simulink model "INC"  (R2020b)
settings: Solver=FixedStepAuto  StartTime=0.0  StopTime=10  FixedStep=1e-2  RelTol=1e-3
libraries: powerlib x1
settings Model: Creator=flocment  LastModifiedBy=bergeslo

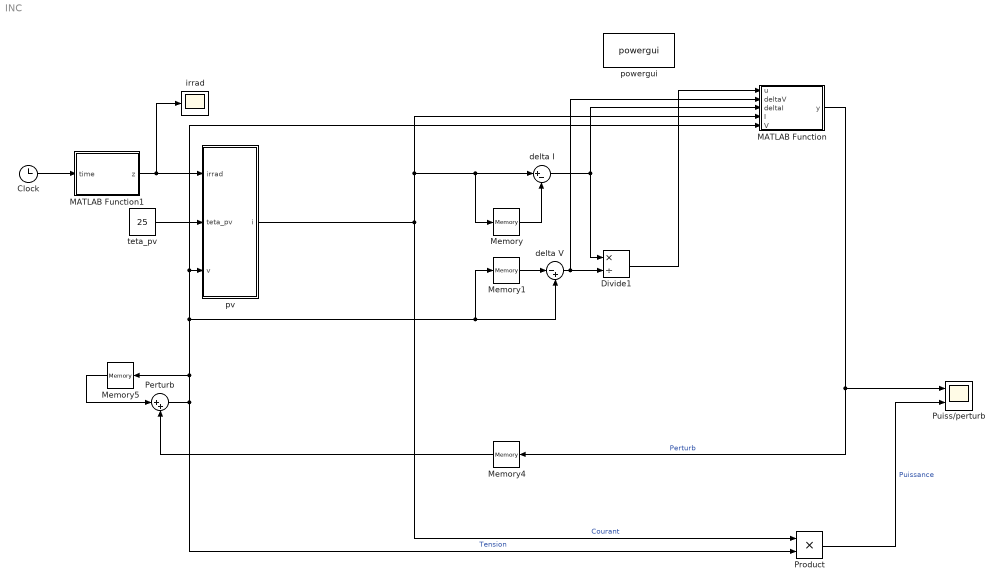
== system INC ==
  Clock : Clock
  Divide1 : Product  Inputs=*/
  MATLAB Function : MATLAB Function  TreatAsAtomicUnit=on
  MATLAB Function1 : MATLAB Function  TreatAsAtomicUnit=on
  Memory : Memory
  Memory1 : Memory
  Memory4 : Memory
  Memory5 : Memory  InitialCondition=5
  Perturb : Sum  Inputs=|++
  Product : Product
  Puiss/perturb : Scope  NumInputPorts=2
  delta I : Sum  Inputs=|+-
  delta V : Sum  Inputs=|-+
  irrad : Scope
  powergui : powerlib/powergui  Priority=1  SimulationMode=Continuous  SampleTime=50e-6  frequency=60  Iterations=50  frequencyindice=60  Pbase=100e6  ErrMax=1e-4  UnitsV=kV  UnitsW=MW  buscounter=0  FunctionMessages=off  echomessages=off  EnableUseOfTLC=off  CurrentSourceSwitches=off  DisableSnubberDevices=off  DisableRonSwitches=off  DisableVfSwitches=off  DisplayEquations=off  AutomaticDiscreteSolvers=off  SolverType=Tustin/Backward Euler (TBE)  Interpol=off  ExternalGateDelay=off  methode=off  Ts=100  x0status=blocks  SPID=on  SwTol=0  HookPort=off  NonlinearTolerance=1e-4  nMaxIteration=100  ContinueOnMaxIteration=off  RestoreLinks=warning  ResistiveCurrentMeasurement=off  Frange=[0:2:500]  Ylog=off  Xlog=on  ShowGrid=off  save=off  variable=ZData  structure=0  ZoomFFT=off  StartTime=0.0  cycles=1  DisplayStyle=1  fundamental=60  FreqAxis=off  MaxFrequency=1000  frequencyindicesteady=1  RmsSteady=1  display=off
  pv : Subsystem
  teta_pv : Constant  Value=25
  wires:
  teta_pv/1 -> pv/2(teta_pv)
  pv/1(i) -> Memory/1, delta I/1, MATLAB Function/4(I), Product/1  "Courant"
  Memory/1 -> delta I/2
  delta I/1 -> Divide1/1, MATLAB Function/3(deltaI)
  Memory1/1 -> delta V/1
  delta V/1 -> MATLAB Function/2(deltaV), Divide1/2
  Divide1/1 -> MATLAB Function/1(u)
  Memory4/1 -> Perturb/2
  Memory5/1 -> Perturb/1
  Perturb/1 -> Product/2, delta V/2, Memory1/1, MATLAB Function/5(V), pv/3(v), Memory5/1  "Tension"
  MATLAB Function/1(y) -> Puiss/perturb/1, Memory4/1  "Perturb"
  Product/1 -> Puiss/perturb/2  "Puissance"
  Clock/1 -> MATLAB Function1/1(time)
  MATLAB Function1/1(z) -> pv/1(irrad), irrad/1

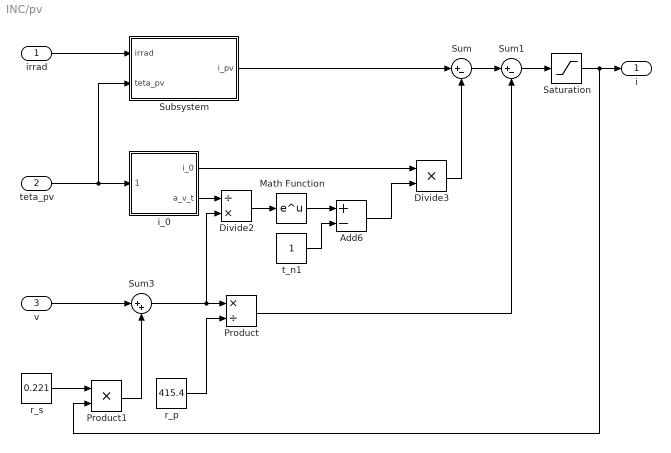
== system INC/pv ==
  irrad : Inport
  teta_pv : Inport  Port=2
  v : Inport  Port=3
  Add6 : Sum  Inputs=+-
  Divide2 : Product  Inputs=/*
  Divide3 : Product  Inputs=**
  Math Function : Math  SaturateOnIntegerOverflow=on
  Product : Product  Inputs=*/
  Product1 : Product
  Saturation : Saturate  UpperLimit=inf  LowerLimit=0
  Subsystem : Subsystem
  Sum : Sum  Inputs=|+-
  Sum1 : Sum  Inputs=|+-
  Sum3 : Sum  Inputs=|++
  i_0 : Subsystem
  r_p : Constant  Value=415.4
  r_s : Constant  Value=0.221
  t_n1 : Constant
  i : Outport
  wires:
  Add6/1 -> Divide3/2
  Sum3/1 -> Divide2/2, Product/1
  Subsystem/1(i_pv) -> Sum/1
  irrad/1 -> Subsystem/1(irrad)
  teta_pv/1 -> Subsystem/2(teta_pv), i_0/1(teta_pv)
  Product1/1 -> Sum3/2
  v/1 -> Sum3/1
  Sum/1 -> Sum1/1
  i_0/1(i_0) -> Divide3/1
  Divide2/1 -> Math Function/1
  i_0/2(a_v_t) -> Divide2/1
  r_p/1 -> Product/2
  r_s/1 -> Product1/1
  t_n1/1 -> Add6/2
  Math Function/1 -> Add6/1
  Sum1/1 -> Saturation/1
  Product/1 -> Sum1/2
  Divide3/1 -> Sum/2
  Saturation/1 -> i/1, Product1/2

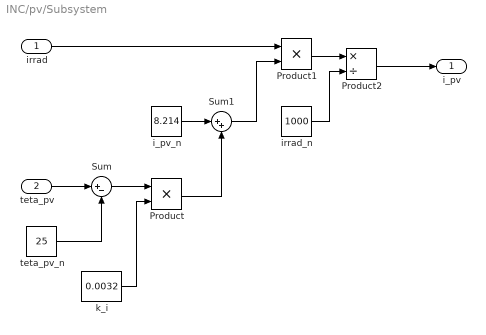
== system INC/pv/Subsystem ==
  irrad : Inport
  teta_pv : Inport  Port=2
  Product : Product
  Product1 : Product
  Product2 : Product  Inputs=*/
  Sum : Sum  Inputs=|+-
  Sum1 : Sum  Inputs=|++
  i_pv_n : Constant  Value=8.214
  irrad_n : Constant  Value=1000
  k_i : Constant  Value=0.0032
  teta_pv_n : Constant  Value=25
  i_pv : Outport
  wires:
  Sum1/1 -> Product1/2
  Product2/1 -> i_pv/1
  teta_pv_n/1 -> Sum/2
  Product1/1 -> Product2/1
  irrad_n/1 -> Product2/2
  Product/1 -> Sum1/2
  i_pv_n/1 -> Sum1/1
  irrad/1 -> Product1/1
  teta_pv/1 -> Sum/1
  k_i/1 -> Product/2
  Sum/1 -> Product/1

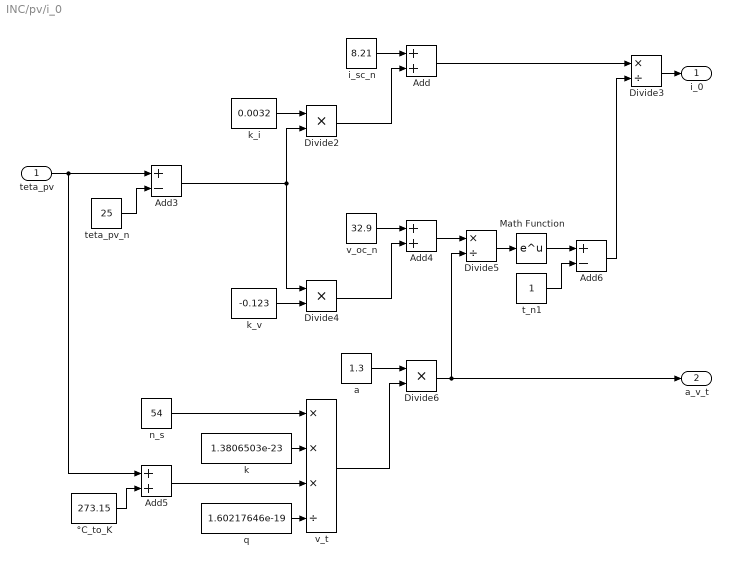
== system INC/pv/i_0 ==
  teta_pv : Inport
  Add : Sum
  Add3 : Sum  Inputs=+-
  Add4 : Sum
  Add5 : Sum
  Add6 : Sum  Inputs=+-
  Divide2 : Product  Inputs=**
  Divide3 : Product  Inputs=*/
  Divide4 : Product  Inputs=**
  Divide5 : Product  Inputs=*/
  Divide6 : Product  Inputs=**
  Math Function : Math  SaturateOnIntegerOverflow=on
  a : Constant  Value=1.3
  i_sc_n : Constant  Value=8.21
  k : Constant  Value=1.3806503e-23
  k_i : Constant  Value=0.0032
  k_v : Constant  Value=-0.123
  n_s : Constant  Value=54
  q : Constant  Value=1.60217646e-19
  t_n1 : Constant
  teta_pv_n : Constant  Value=25
  v_oc_n : Constant  Value=32.9
  v_t : Product  Inputs=***/
  °C_to_K : Constant  Value=273.15
  i_0 : Outport
  a_v_t : Outport  Port=2
  wires:
  Divide3/1 -> i_0/1
  Add4/1 -> Divide5/1
  Add/1 -> Divide3/1
  q/1 -> v_t/4
  k_v/1 -> Divide4/2
  k/1 -> v_t/2
  Divide5/1 -> Math Function/1
  Add5/1 -> v_t/3
  Divide6/1 -> a_v_t/1, Divide5/2
  Math Function/1 -> Add6/1
  Add6/1 -> Divide3/2
  v_t/1 -> Divide6/2
  Add3/1 -> Divide4/1, Divide2/2
  n_s/1 -> v_t/1
  teta_pv/1 -> Add5/1, Add3/1
  Divide4/1 -> Add4/2
  v_oc_n/1 -> Add4/1
  a/1 -> Divide6/1
  t_n1/1 -> Add6/2
  Divide2/1 -> Add/2
  teta_pv_n/1 -> Add3/2
  i_sc_n/1 -> Add/1
  k_i/1 -> Divide2/1
  °C_to_K/1 -> Add5/2

== matlab function INC/MATLAB Function1 ==
  data: time input; z output
function z = fcn(time)
    if time<2
    z=400;
    elseif 2<time && time<5
    z=800;
    else
    z=300;
    end

== matlab function INC/MATLAB Function ==
  data: u input; y output; deltaV input; deltaI input; I input; V input
function y = fcn(u, deltaV, deltaI, I, V)
if deltaV==0

    if deltaI>0
    y=1;
    elseif deltaI<0
    y=-1;
    else
    y=0;
    end

else
j=I+u*V;

   if j>0
   y=1;
   elseif j<0
   y=-1;
   else
   y=0;
   end
end   
end
